simulink model "Simulaciones_de_Control"  (R2026b)
settings: Solver=ode15s  StopTime=3  MaxStep=1e-3
values from neighbouring files (symbols this model uses):
  alpha_Cu = 3.9e-3    (= 0.0039)    [coeficientes.m]
  b_eq = b_m + b_l/(r^2)    (= 2.19444444444e-05)    [coeficientes.m]
  C_ts = 0.818    [coeficientes.m]
  g = 9.80665    [coeficientes.m]
  init_I0 = 0    [coeficientes.m]
  init_Id = 0    [coeficientes.m]
  init_Iq = 0    [coeficientes.m]
  init_theta = 0    [coeficientes.m]
  init_Ts = 20    [coeficientes.m]
  init_w = 0    [coeficientes.m]
  J_eq = J_m + J_l/(r^2)    (= 4.58263888889e-05)    [coeficientes.m]
  K_et = 2*p_obs    (= 6400)    [coeficientes.m]
  K_ew = p_obs^2    (= 10240000)    [coeficientes.m]
  k_l = k_l_min + m_l*l_l    (= 1)    [coeficientes.m]
  Kd_mov = wn_mov * (2*zeta_mov + 1) * J_eq    (= 0.0916527777778)    [coeficientes.m]
  Ki_mov = wn_mov^3 * J_eq    (= 23463.1111111)    [coeficientes.m]
  Kp_mov = wn_mov^2 * (2*zeta_mov + 1) * J_eq    (= 73.3222222222)    [coeficientes.m]
  L_d = 6.6e-3    (= 0.0066)    [coeficientes.m]
  L_ls = 0.8e-3    (= 0.0008)    [coeficientes.m]
  L_q = 5.8e-3    (= 0.0058)    [coeficientes.m]
  lambda = 0.016    [coeficientes.m]
  Pp = 3    [coeficientes.m]
  r = 120.0    (= 120)    [coeficientes.m]
  R_sREF = 1.02    [coeficientes.m]
  R_tsamb = 146.7    [coeficientes.m]
  T_amb = 20    [coeficientes.m]
  T_sREF = 20    [coeficientes.m]
libraries: eeTransforms x12
(part 1 of 2)
settings Model: Creator=fedeb  LastModifiedBy=fedeb
settings SimscapeCC: SimscapeLogType=all  SimscapeNominalValues="[{\"value\":\"1\",\"unit\":\"A\"},{\"value\":\"1\",\"unit\":\"bar\"},{\"value\":\"1\",\"unit\":\"cm^2\"},{\"value\":\"1\",\"unit\":\"cm^3/s\"},{\"value\":\"1\",\"unit\":\"kJ/kg\"},{\"value\":\"1\",\"unit\":\"kW\"},{\"value\":\"1\",\"unit\":\"l\"},{\"value\":\"1\",\"unit\":\"N\"},{\"value\":\"1\",\"unit\":\"N*m\"},{\"value\":\"1\",\"unit\":\"V\"},{\"value\":\"0.001\",\"unit\":\"Wb\"}]"  SimscapeUseEnergyAccounting=off

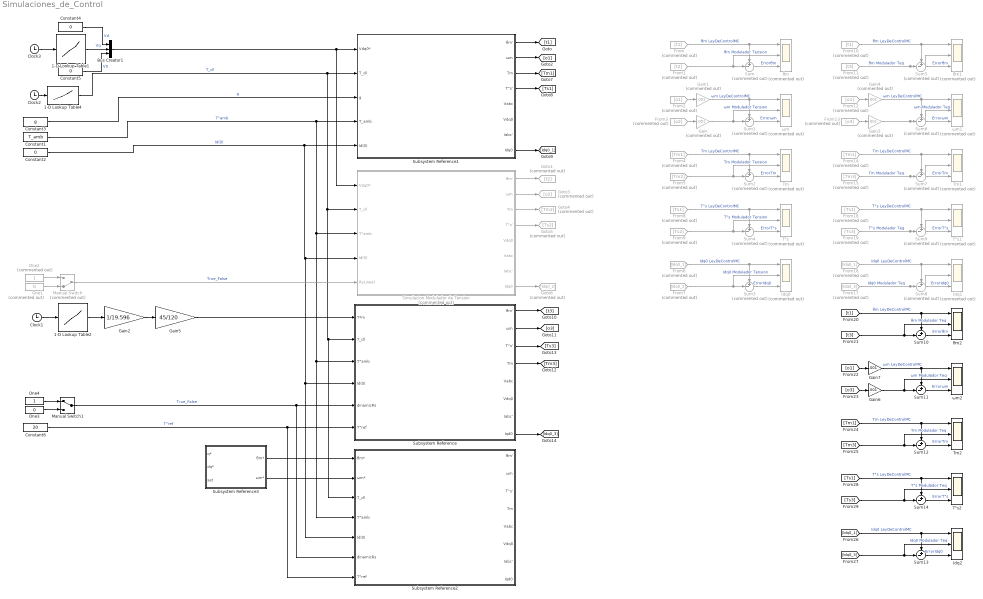
== system Simulaciones_de_Control ==
  1-D Lookup Table1 : Lookup_n-D  NumberOfTableDimensions=1  BreakpointsForDimension1=[0.0, 0.1, 0.101, 0.3, 0.301, 0.5, 0.501, 0.7, 0.701, 0.9, 0.901, 1.1, 1.101, 1.3, 1.301, 1.5, 1.501, 1.7, 1.701, 1.9, 1.901, 2.0]  Table=[0.0, 0.0, 19.596, 19.596, 19.596, 19.596, 19.596, 19.596, 0.0, 0.0, 0.0, 0.0, -19.596, -19.596, -19.596, -19.596, -19.596, -19.596, 0.0, 0.0, 0.0, 0.0]  InternalRulePriority=Speed  RndMeth=Simplest
  1-D Lookup Table2 : Lookup_n-D  NumberOfTableDimensions=1  BreakpointsForDimension1=[0.0, 0.1, 0.101, 0.3, 0.301, 0.5, 0.501, 0.7, 0.701, 0.9, 0.901, 1.1, 1.101, 1.3, 1.301, 1.5, 1.501, 1.7, 1.701, 1.9, 1.901, 2.0]  Table=[0.0, 0.0, 19.596, 19.596, 19.596, 19.596, 19.596, 19.596, 0.0, 0.0, 0.0, 0.0, -19.596, -19.596, -19.596, -19.596, -19.596, -19.596, 0.0, 0.0, 0.0, 0.0]  InternalRulePriority=Speed  RndMeth=Simplest
  1-D Lookup Table4 : Lookup_n-D  NumberOfTableDimensions=1  BreakpointsForDimension1=[0.0, 0.1, 0.101, 0.3, 0.301, 0.5, 0.501, 0.7, 0.701, 0.9, 0.901, 1.1, 1.101, 1.3, 1.301, 1.5, 1.501, 1.7, 1.701, 1.9, 1.901, 2.0]  Table=[0.0, 0.0, 0.0, 0.0, 6.28, 6.28, -6.28, -6.28, -6.28, -6.28, 0.0, 0.0, 0.0, 0.0, 6.28, 6.28, -6.28, -6.28, 0.0, 0.0, 0.0, 0.0]  InternalRulePriority=Speed  RndMeth=Simplest
  Bus Creator1 : BusCreator  Inputs=3
  Clock1 : Clock
  Clock2 : Clock
  Clock3 : Clock
  Constant1 : Constant  Value=T_amb
  Constant2 : Constant  Value=0
  Constant3 : Constant  Value=g
  Constant4 : Constant  Value=0
  Constant5 : Constant  Value=0
  Constant6 : Constant  Value=20
  From : From  Commented=on  GotoTag=t1
  From1 : From  Commented=on  GotoTag=t2
  From10 : From  Commented=on  GotoTag=t1
  From11 : From  Commented=on  GotoTag=t3
  From12 : From  Commented=on  GotoTag=o1
  From13 : From  Commented=on  GotoTag=o3
  From14 : From  Commented=on  GotoTag=Tm1
  From15 : From  Commented=on  GotoTag=Tm3
  From16 : From  Commented=on  GotoTag=Idq0_1
  From17 : From  Commented=on  GotoTag=Idq0_3
  From18 : From  Commented=on  GotoTag=Ts1
  From19 : From  Commented=on  GotoTag=Ts3
  From2 : From  Commented=on  GotoTag=o1
  From3 : From  Commented=on  GotoTag=o2
  From4 : From  Commented=on  GotoTag=Tm1
  From5 : From  Commented=on  GotoTag=Tm2
  From6 : From  Commented=on  GotoTag=Idq0_1
  From7 : From  Commented=on  GotoTag=Idq0_2
  From8 : From  Commented=on  GotoTag=Ts1
  From9 : From  Commented=on  GotoTag=Ts2
  Gain{,1,3..4} (4 alike) : Gain  Commented=on  Gain=.001
  Gain2 : Gain  Gain=1/19.596
  Gain5 : Gain  Gain=45/120
  Gain6 : Gain  Gain=.001
  Gain7 : Gain  Gain=.001
  Goto1 : Goto  Commented=on  GotoTag=t2
  Goto3 : Goto  Commented=on  GotoTag=o2
  Goto4 : Goto  Commented=on  GotoTag=Tm2
  Goto5 : Goto  Commented=on  GotoTag=Ts2
  Goto6 : Goto  Commented=on  GotoTag=Idq0_2
  Idq0 : Scope  Commented=on  NumInputPorts=3
      settings: Title=Comparación Idq0  ActiveDisplayYMinimum=-22.799596876170931  ActiveDisplayYMaximum=77.542210763995357  YLabel=Idq0 [A]  DataLoggingVariableName=ScopeData3
  Idq1 : Scope  Commented=on  NumInputPorts=3
      settings: Title=Comparación Idq0  ActiveDisplayYMinimum=-15.292921358243067  ActiveDisplayYMaximum=15.917825301373405  YLabel=Idq0 [A]  DataLoggingVariableName=ScopeData4
  Idq2 : Scope  NumInputPorts=3
      settings: Title=Comparación Idq0  ActiveDisplayYMinimum=-15.292921358243067  ActiveDisplayYMaximum=15.917825301373405  YLabel=Idq0 [A]  DataLoggingVariableName=ScopeData10
  Manual Switch : ManualSwitch  Commented=on  CurrentSetting=0
  Manual Switch1 : ManualSwitch
  One1 : Constant  Commented=on  Value=0  OutDataTypeStr=Inherit: Inherit via back propagation
  One2 : Constant  Commented=on  OutDataTypeStr=Inherit: Inherit via back propagation
  One3 : Constant  Value=0  OutDataTypeStr=Inherit: Inherit via back propagation
  One4 : Constant  OutDataTypeStr=Inherit: Inherit via back propagation
  Simulacion Modulador de Tension : Subsystem  Commented=on
  Subsystem Reference : Subsystem
  Subsystem Reference1 : Subsystem
  Subsystem Reference2 : Subsystem
  Subsystem Reference3 : Subsystem
  Sum{,1..9} (10 alike) : Sum  Commented=on  Inputs=+-|
  Sum{10..14} (5 alike) : Sum  Inputs=+-|
  Tm : Scope  Commented=on  NumInputPorts=3
      settings: Title=Comparación Torque Motor  ActiveDisplayYMinimum=-1.641570975092526  ActiveDisplayYMaximum=5.5830391750086239  YLabel=T_m [Nm]
  Tm1 : Scope  Commented=on  NumInputPorts=3
      settings: Title=Comparación Torque Motor  ActiveDisplayYMinimum=-1.1010903377934618  ActiveDisplayYMaximum=1.1460834216988809  YLabel=T_m [Nm]  DataLoggingVariableName=ScopeData6
  Tm2 : Scope  NumInputPorts=3
      settings: Title=Comparación Torque Motor  ActiveDisplayYMinimum=-1.1010903377934618  ActiveDisplayYMaximum=1.1460834216988809  YLabel=T_m [Nm]  DataLoggingVariableName=ScopeData11
  T°s : Scope  Commented=on  NumInputPorts=3
      settings: Title=Comparación θm  ActiveDisplayYMinimum=-1017.2983087504352  ActiveDisplayYMaximum=1033.0305039187574  DataLoggingVariableName=ScopeData2
  T°s1 : Scope  Commented=on  NumInputPorts=3
      settings: Title=Comparación T°s  ActiveDisplayYMinimum=10.145079259650506  ActiveDisplayYMaximum=108.69428666314548  YLabel=T°s [°C]  DataLoggingVariableName=ScopeData7
  T°s2 : Scope  NumInputPorts=3
      settings: Title=Comparación T°s  ActiveDisplayYMinimum=10.145079259650506  ActiveDisplayYMaximum=108.69428666314548  YLabel=T°s [°C]  DataLoggingVariableName=ScopeData12
  θm : Scope  Commented=on  NumInputPorts=3
      settings: Title=Comparación θm  ActiveDisplayYMinimum=-15548.638838676963  ActiveDisplayYMaximum=15530.228334297437
  θm1 : Scope  Commented=on  NumInputPorts=3
      settings: Title=Comparación θm  ActiveDisplayYMinimum=-693.83102797369031  ActiveDisplayYMaximum=5988.9336809294882  YLabel=\theta_m [rad]  DataLoggingVariableName=ScopeData8
  θm2 : Scope  NumInputPorts=3
      settings: Title=Comparación θm  ActiveDisplayYMinimum=-693.83102797369031  ActiveDisplayYMaximum=5988.9336809294882  YLabel=\theta_m [rad]  DataLoggingVariableName=ScopeData13
  ωm : Scope  Commented=on  NumInputPorts=3
      settings: Title=Comparación ωm  ActiveDisplayYMinimum=-1.8612728525157345  ActiveDisplayYMaximum=12.323556548165303  YLabel=\omega_{motor} [10^3 rad/s]  DataLoggingVariableName=ScopeData5
  ωm1 : Scope  Commented=on  NumInputPorts=3
      settings: Title=Comparación ωm  ActiveDisplayYMinimum=-1.1427898971415431  ActiveDisplayYMaximum=5.8360821110076726  YLabel=\omega_{motor} [10^3 rad/s]  DataLoggingVariableName=ScopeData9
  ωm2 : Scope  NumInputPorts=3
      settings: Title=Comparación ωm  ActiveDisplayYMinimum=-1.1427898971415431  ActiveDisplayYMaximum=5.8360821110076726  YLabel=\omega_{motor} [10^3 rad/s]  DataLoggingVariableName=ScopeData14
  wires:
  Clock3/1 -> 1-D Lookup Table1/1
  1-D Lookup Table1/1 -> Bus Creator1/2  "Vq"
  Clock2/1 -> 1-D Lookup Table4/1
  Constant5/1 -> Bus Creator1/3  "V0"
  Constant4/1 -> Bus Creator1/1  "Vd"
  1-D Lookup Table4/1 -> Subsystem Reference2/3(T_dl), Subsystem Reference/2(T_dl), Simulacion Modulador de Tension/2(T_dl), Subsystem Reference1/2(T_dl)  "T_dl"
  Bus Creator1/1 -> Simulacion Modulador de Tension/1(Vdq0*), Subsystem Reference1/1(Vdq0*)
  Constant3/1 -> Subsystem Reference1/3(g)  "g"
  Constant1/1 -> Subsystem Reference2/4(T°amb), Subsystem Reference/3(T°amb), Simulacion Modulador de Tension/3(T°amb), Subsystem Reference1/4(T_amb)  "T°amb"
  Constant2/1 -> Subsystem Reference2/5(Id(0)), Subsystem Reference/4(Id(0)), Simulacion Modulador de Tension/4(Id(0)), Subsystem Reference1/5(Id(0))  "Id(0)"
  One2/1 -> Manual Switch/1
  One1/1 -> Manual Switch/2
  Manual Switch/1 -> Simulacion Modulador de Tension/5(RsLineal)  "True_False"
  Sum/1 -> θm/3  "Errorθm"
  Subsystem Reference1/1(θm') -> [t1]
  From/1 -> θm/1, Sum/1  "θm LeyDeControlMC"
  Simulacion Modulador de Tension/1(θm') -> Goto1/1
  From1/1 -> θm/2, Sum/2  "θm Modulador Tension"
  From3/1 -> Gain/1
  Sum1/1 -> ωm/3  "Errorωm"
  From2/1 -> Gain1/1
  From5/1 -> Tm/2, Sum2/2  "Tm Modulador Tension"
  Sum2/1 -> Tm/3  "ErrorTm"
  From4/1 -> Tm/1, Sum2/1  "Tm LeyDeControlMC"
  From7/1 -> Idq0/2, Sum3/2  "Idq0 Modulador Tension"
  Sum3/1 -> Idq0/3  "ErrorIdq0"
  From6/1 -> Idq0/1, Sum3/1  "Idq0 LeyDeControlMC"
  Subsystem Reference1/2(ωm) -> [o1]
  Subsystem Reference1/3(Tm) -> [Tm1]
  Subsystem Reference1/4(T°s') -> [Ts1]
  Subsystem Reference1/8(Idq0) -> [Idq0_1]
  Simulacion Modulador de Tension/2(ωm) -> Goto3/1
  Simulacion Modulador de Tension/3(Tm) -> Goto4/1
  Simulacion Modulador de Tension/4(T°s') -> Goto5/1
  Simulacion Modulador de Tension/8(Idq0) -> Goto6/1
  From8/1 -> T°s/1, Sum4/1  "T°s LeyDeControlMC"
  Sum4/1 -> T°s/3  "ErrorT°s"
  From9/1 -> T°s/2, Sum4/2  "T°s Modulador Tension"
  Gain/1 -> ωm/2, Sum1/2  "ωm Modulador Tension"
  Gain1/1 -> ωm/1, Sum1/1  "ωm LeyDeControlMC"
  Subsystem Reference/1(θm') -> [t3]
  Clock1/1 -> 1-D Lookup Table2/1
  1-D Lookup Table2/1 -> Gain2/1
  Gain2/1 -> Gain5/1
  One4/1 -> Manual Switch1/1
  One3/1 -> Manual Switch1/2
  Manual Switch1/1 -> Subsystem Reference2/6(dinamicRs), Subsystem Reference/5(dinamicRs)  "True_False"
  Constant6/1 -> Subsystem Reference2/7(T°ref), Subsystem Reference/6(T°ref)  "T°ref"
  Subsystem Reference/2(ωm) -> [o3]
  Subsystem Reference/3(T°s') -> [Ts3]
  Subsystem Reference/4(Tm) -> [Tm3]
  Subsystem Reference/8(Iqd0) -> [Idq0_3]
  Sum9/1 -> T°s1/3  "ErrorT°s"
  Sum6/1 -> ωm1/3  "Errorωm"
  From16/1 -> Idq1/1, Sum8/1  "Idq0 LeyDeControlMC"
  From19/1 -> T°s1/2, Sum9/2  "T°s Modulador Teq"
  Gain3/1 -> ωm1/2, Sum6/2  "ωm Modulador Teq"
  From14/1 -> Tm1/1, Sum7/1  "Tm LeyDeControlMC"
  Gain4/1 -> ωm1/1, Sum6/1  "ωm LeyDeControlMC"
  Sum7/1 -> Tm1/3  "ErrorTm"
  From17/1 -> Idq1/2, Sum8/2  "Idq0 Modulador Teq"
  Sum8/1 -> Idq1/3  "ErrorIdq0"
  From12/1 -> Gain4/1
  From11/1 -> θm1/2, Sum5/2  "θm Modulador Teq"
  From18/1 -> T°s1/1, Sum9/1  "T°s LeyDeControlMC"
  Sum5/1 -> θm1/3  "Errorθm"
  From10/1 -> θm1/1, Sum5/1  "θm LeyDeControlMC"
  From13/1 -> Gain3/1
  From15/1 -> Tm1/2, Sum7/2  "Tm Modulador Teq"
  Gain5/1 -> Subsystem Reference/1(T*m)
  [Idq0_1] -> Idq2/1, Sum13/1  "Idq0 LeyDeControlMC"
  [Ts3] -> T°s2/2, Sum14/2  "T°s Modulador Teq"
  Sum10/1 -> θm2/3  "Errorθm"
  [t1] -> θm2/1, Sum10/1  "θm LeyDeControlMC"
  Sum14/1 -> T°s2/3  "ErrorT°s"
  [Idq0_3] -> Idq2/2, Sum13/2  "Idq0 Modulador Teq"
  Sum11/1 -> ωm2/3  "Errorωm"
  [t3] -> θm2/2, Sum10/2  "θm Modulador Teq"
  Sum12/1 -> Tm2/3  "ErrorTm"
  [Ts1] -> T°s2/1, Sum14/1  "T°s LeyDeControlMC"
  [Tm1] -> Tm2/1, Sum12/1  "Tm LeyDeControlMC"
  Gain7/1 -> ωm2/1, Sum11/1  "ωm LeyDeControlMC"
  [Tm3] -> Tm2/2, Sum12/2  "Tm Modulador Teq"
  [o1] -> Gain7/1
  Gain6/1 -> ωm2/2, Sum11/2  "ωm Modulador Teq"
  [o3] -> Gain6/1
  Sum13/1 -> Idq2/3  "ErrorIdq0"
  Subsystem Reference3/2(ωm*) -> Subsystem Reference2/2(ωm*)
  Subsystem Reference3/1(θm*) -> Subsystem Reference2/1(θm*)

== system Simulaciones_de_Control/Simulacion Modulador de Tension ==
  Vdq0* : Inport  OutDataTypeStr=Bus: Vdq0
  T_dl : Inport  Port=2
  T°amb : Inport  Port=3
  Id(0) : Inport  Port=4
  RsLineal : Inport  Port=5
  Bus Selector2 : BusSelector  OutputSignals=Vd,Vq,V0
  Constant : Constant  Value=g
  Constant2 : Constant  Value=R_sREF
  Modulador de Tensiones Virtuales : Subsystem
      settings: PortSchema="{\"entries\":[{\"content\":{\"sides\":[{\"content\":{\"connectorIds\":[\"In2\",\"In1\",\"In3\",\"In6\",\"In7\",\"In5\",\"In4\"]},\"type\":\"ConnectorPlacement.EquallySpacedRectSide\",\"uuid\":\"561a625a-719f-47d4-85d3-a88e423068dd\"},{\"content\":{\"connectorIds\":[\"Out2\",\"Out1\"],\"side\":\"RIGHT\"},\"type\":\"ConnectorPlacement.EquallySpacedRectSide\",\"uuid\":\"c1cdd74a-6c1d-470e-a6ac-8d72e83b5cc5\"},{\"content\":{\"side\":\"TOP\"},\"type\":\"ConnectorPlacement.EquallySpacedRectSide\",\"uuid\":\"c5935c6f-534c-46b9-aa64-6d6dabbbb210\"}]},\"type\":\"ConnectorPlacement.EquallySpacedConnector\",\"uuid\":\"b0debde9-6e18-4e06-b0c4-28c9c51e472d\"}],\"packageUris\":[\"http://schema.mathworks.com/mf0/Connector/R2020b\"],\"version\":\"1.0\"}"
  Planta (Modelo Global No Lineal) : Subsystem
      settings: PortSchema="{\"entries\":[{\"content\":{\"sides\":[{\"content\":{\"connectorIds\":[\"In1\",\"In3\",\"In2\",\"In4\",\"In5\"]},\"type\":\"ConnectorPlacement.EquallySpacedRectSide\",\"uuid\":\"3481abf0-b0cb-49f6-b93f-5a31fbfa4119\"},{\"content\":{\"connectorIds\":[\"Out1\",\"Out2\",\"Out3\",\"Out4\",\"Out5\"],\"side\":\"RIGHT\"},\"type\":\"ConnectorPlacement.EquallySpacedRectSide\",\"uuid\":\"81dbc61e-d5f3-4edc-bc73-ec3d6160a008\"},{\"content\":{\"side\":\"TOP\"},\"type\":\"ConnectorPlacement.EquallySpacedRectSide\",\"uuid\":\"48e37594-92fb-4835-b4aa-9211b8b6a309\"}]},\"type\":\"ConnectorPlacement.EquallySpacedConnector\",\"uuid\":\"6c32b8e1-5803-41f4-af4e-ba3a494349ba\"}],\"packageUris\":[\"http://schema.mathworks.com/mf0/Connector/R2020b\"],\"version\":\"1.0\"}"
  Sensores Ideales : Subsystem
      settings: PortSchema="{\"entries\":[{\"content\":{\"sides\":[{\"content\":{\"connectorIds\":[\"In1\",\"In2\",\"In3\"]},\"type\":\"ConnectorPlacement.EquallySpacedRectSide\",\"uuid\":\"f4bb6189-c8cb-4d3e-a45f-895d59b6a7f9\"},{\"content\":{\"connectorIds\":[\"Out3\",\"Out2\",\"Out1\"],\"side\":\"RIGHT\"},\"type\":\"ConnectorPlacement.EquallySpacedRectSide\",\"uuid\":\"4fe23da4-d7b3-4116-8a5c-3a889a14c1ed\"},{\"content\":{\"side\":\"TOP\"},\"type\":\"ConnectorPlacement.EquallySpacedRectSide\",\"uuid\":\"3a675bb7-2a54-45fb-91cd-5f3dc1d0d742\"}]},\"type\":\"ConnectorPlacement.EquallySpacedConnector\",\"uuid\":\"fa703284-8060-4ab8-a349-fe5cb05f502a\"}],\"packageUris\":[\"http://schema.mathworks.com/mf0/Connector/R2020b\"],\"version\":\"1.0\"}"
  Subsystem : Subsystem
  Switch : Switch  Criteria=u2 > Threshold  SaturateOnIntegerOverflow=off  InputSameDT=off
  Transformada_Directa_de_Park_I : Subsystem
  θm' : Outport
  ωm : Outport  Port=2
  Tm : Outport  Port=3
  T°s' : Outport  Port=4
  Vdq0 : Outport  Port=5
  Vabc : Outport  Port=6
  Iabc' : Outport  Port=7
  Idq0 : Outport  Port=8  OutDataTypeStr=Bus: Idq0
  wires:
  Planta (Modelo Global No Lineal)/5(Tm) -> Tm/1
  Id(0)/1 -> Planta (Modelo Global No Lineal)/5(Id(0))
  T_dl/1 -> Planta (Modelo Global No Lineal)/2(T_ld)
  Modulador de Tensiones Virtuales/2(Vdq0) -> Vdq0/1
  Planta (Modelo Global No Lineal)/3(T°s) -> Sensores Ideales/3(T°s)
  Sensores Ideales/2(Iabc') -> Transformada_Directa_de_Park_I/1(Iabc), Modulador de Tensiones Virtuales/6(Iabc), Iabc'/1  "Iabc'"
  T°amb/1 -> Planta (Modelo Global No Lineal)/4(T°amb)
  Constant/1 -> Planta (Modelo Global No Lineal)/3(g)
  Planta (Modelo Global No Lineal)/1(θm) -> Sensores Ideales/1(θm)
  Modulador de Tensiones Virtuales/1(Vabc) -> Vabc/1, Planta (Modelo Global No Lineal)/1(Vabc)
  Sensores Ideales/3(T°s') -> Subsystem/1(T°s), T°s'/1  "T°s'"
  Sensores Ideales/1(θm') -> Transformada_Directa_de_Park_I/2(θm), Modulador de Tensiones Virtuales/7(θm), θm'/1  "θm'"
  Planta (Modelo Global No Lineal)/2(Iabc) -> Sensores Ideales/2(Iabc)
  Planta (Modelo Global No Lineal)/4(ωm) -> Modulador de Tensiones Virtuales/5(ωm), ωm/1  "ωm"
  Subsystem/1(R_s) -> Switch/1  "Rs"
  RsLineal/1 -> Switch/2  "True_False"
  Switch/1 -> Modulador de Tensiones Virtuales/4(Rs)  "Rs"
  Constant2/1 -> Switch/3
  Transformada_Directa_de_Park_I/1(Idq0) -> Idq0/1
  Bus Selector2/1 -> Modulador de Tensiones Virtuales/2(Vd*)  "<Vd>"
  Bus Selector2/3 -> Modulador de Tensiones Virtuales/3(V0*)  "<V0>"
  Bus Selector2/2 -> Modulador de Tensiones Virtuales/1(Vq*)  "<Vq>"
  Vdq0*/1 -> Bus Selector2/1

== system Simulaciones_de_Control/Subsystem Reference ==
  T*m : Inport
  T_dl : Inport  Port=2
  T°amb : Inport  Port=3
  Id(0) : Inport  Port=4
  dinamicRs : Inport  Port=5
  T°ref : Inport  Port=6
  Constant : Constant  Value=g
  Modulador de Torque Equivalente : Subsystem
      settings: PortSchema="{\"entries\":[{\"content\":{\"sides\":[{\"content\":{\"connectorIds\":[\"In1\",\"In3\",\"In5\",\"In2\",\"In4\",\"In6\",\"In7\"]},\"type\":\"ConnectorPlacement.EquallySpacedRectSide\",\"uuid\":\"ea9ad4ab-f607-4d37-9442-85f6cfda2486\"},{\"content\":{\"connectorIds\":[\"Out2\",\"Out1\"],\"side\":\"RIGHT\"},\"type\":\"ConnectorPlacement.EquallySpacedRectSide\",\"uuid\":\"696b5fe5-1f6c-4fc9-932e-86b56d49996f\"},{\"content\":{\"side\":\"TOP\"},\"type\":\"ConnectorPlacement.EquallySpacedRectSide\",\"uuid\":\"45e3ac4c-5a2f-4a79-9454-e497b07295c7\"}]},\"type\":\"ConnectorPlacement.EquallySpacedConnector\",\"uuid\":\"ad401c21-3c60-4ab4-96eb-f449fc93609a\"}],\"packageUris\":[\"http://schema.mathworks.com/mf0/Connector/R2020b\"],\"version\":\"1.0\"}"
  Planta (Modelo Global No Lineal) : Subsystem
      settings: PortSchema="{\"entries\":[{\"content\":{\"sides\":[{\"content\":{\"connectorIds\":[\"In1\",\"In3\",\"In2\",\"In4\",\"In5\"]},\"type\":\"ConnectorPlacement.EquallySpacedRectSide\",\"uuid\":\"3481abf0-b0cb-49f6-b93f-5a31fbfa4119\"},{\"content\":{\"connectorIds\":[\"Out1\",\"Out2\",\"Out3\",\"Out4\",\"Out5\"],\"side\":\"RIGHT\"},\"type\":\"ConnectorPlacement.EquallySpacedRectSide\",\"uuid\":\"81dbc61e-d5f3-4edc-bc73-ec3d6160a008\"},{\"content\":{\"side\":\"TOP\"},\"type\":\"ConnectorPlacement.EquallySpacedRectSide\",\"uuid\":\"48e37594-92fb-4835-b4aa-9211b8b6a309\"}]},\"type\":\"ConnectorPlacement.EquallySpacedConnector\",\"uuid\":\"6c32b8e1-5803-41f4-af4e-ba3a494349ba\"}],\"packageUris\":[\"http://schema.mathworks.com/mf0/Connector/R2020b\"],\"version\":\"1.0\"}"
  Sensores Ideales : Subsystem
      settings: PortSchema="{\"entries\":[{\"content\":{\"sides\":[{\"content\":{\"connectorIds\":[\"In1\",\"In2\",\"In3\"]},\"type\":\"ConnectorPlacement.EquallySpacedRectSide\",\"uuid\":\"f4bb6189-c8cb-4d3e-a45f-895d59b6a7f9\"},{\"content\":{\"connectorIds\":[\"Out3\",\"Out2\",\"Out1\"],\"side\":\"RIGHT\"},\"type\":\"ConnectorPlacement.EquallySpacedRectSide\",\"uuid\":\"4fe23da4-d7b3-4116-8a5c-3a889a14c1ed\"},{\"content\":{\"side\":\"TOP\"},\"type\":\"ConnectorPlacement.EquallySpacedRectSide\",\"uuid\":\"3a675bb7-2a54-45fb-91cd-5f3dc1d0d742\"}]},\"type\":\"ConnectorPlacement.EquallySpacedConnector\",\"uuid\":\"fa703284-8060-4ab8-a349-fe5cb05f502a\"}],\"packageUris\":[\"http://schema.mathworks.com/mf0/Connector/R2020b\"],\"version\":\"1.0\"}"
  Transformada_Directa_de_Park_I : Subsystem
  θm' : Outport
  ωm : Outport  Port=2
  T°s' : Outport  Port=3
  Tm : Outport  Port=4
  Vabc : Outport  Port=5  OutDataTypeStr=Bus: Vabc
  Vdq0 : Outport  Port=6  OutDataTypeStr=Bus: Vdq0
  Iabc' : Outport  Port=7  OutDataTypeStr=Bus: Iabc
  Iqd0 : Outport  Port=8  OutDataTypeStr=Bus: Idq0
  wires:
  Planta (Modelo Global No Lineal)/1(θm) -> Sensores Ideales/1(θm)
  Sensores Ideales/1(θm') -> θm'/1, Transformada_Directa_de_Park_I/2(θm), Modulador de Torque Equivalente/4(θm)  "θm'"
  Planta (Modelo Global No Lineal)/2(Iabc) -> Sensores Ideales/2(Iabc)
  Modulador de Torque Equivalente/1(Vabc) -> Planta (Modelo Global No Lineal)/1(Vabc), Vabc/1
  Planta (Modelo Global No Lineal)/3(T°s) -> Sensores Ideales/3(T°s)
  Sensores Ideales/2(Iabc') -> Transformada_Directa_de_Park_I/1(Iabc), Modulador de Torque Equivalente/3(Iabc), Iabc'/1  "Iabc'"
  Sensores Ideales/3(T°s') -> T°s'/1, Modulador de Torque Equivalente/1(T°s)  "T°s'"
  Constant/1 -> Planta (Modelo Global No Lineal)/3(g)
  Id(0)/1 -> Planta (Modelo Global No Lineal)/5(Id(0))  "Id(0)"
  T°amb/1 -> Planta (Modelo Global No Lineal)/4(T°amb)  "T°amb"
  T_dl/1 -> Planta (Modelo Global No Lineal)/2(T_ld)  "T_dl"
  Planta (Modelo Global No Lineal)/5(Tm) -> Tm/1
  Planta (Modelo Global No Lineal)/4(ωm) -> Modulador de Torque Equivalente/2(ωm), ωm/1
  Modulador de Torque Equivalente/2(Vdq0) -> Vdq0/1
  dinamicRs/1 -> Modulador de Torque Equivalente/6(dinamicRs?)
  T°ref/1 -> Modulador de Torque Equivalente/7(T°ref)
  T*m/1 -> Modulador de Torque Equivalente/5(T*m)  "T*m"
  Transformada_Directa_de_Park_I/1(Idq0) -> Iqd0/1

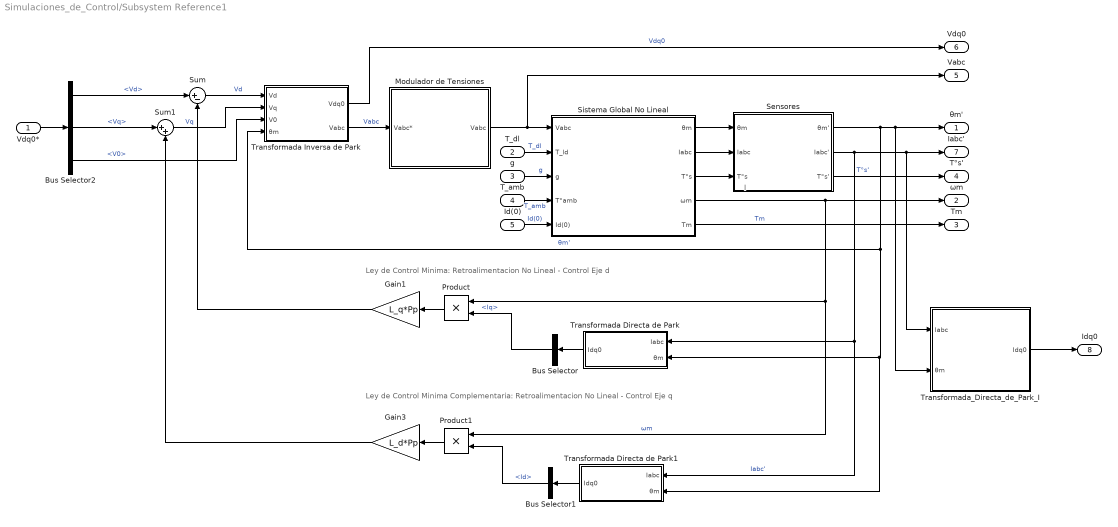
== system Simulaciones_de_Control/Subsystem Reference1 ==
  note: Ley de Control Minima: Retroalimentacion No Lineal - Control Eje d
  note: I
  note: Ley de Control Minima Complementaria: Retroalimentacion No Lineal - Control Eje q
  Vdq0* : Inport  OutDataTypeStr=Bus: Vdq0
  T_dl : Inport  Port=2
  g : Inport  Port=3
  T_amb : Inport  Port=4
  Id(0) : Inport  Port=5
  Bus Selector : BusSelector  OutputSignals=Iq
  Bus Selector1 : BusSelector  OutputSignals=Id
  Bus Selector2 : BusSelector  OutputSignals=Vd,Vq,V0
  Gain1 : Gain  Gain=L_q*Pp
  Gain3 : Gain  Gain=L_d*Pp
  Modulador de Tensiones : Subsystem
  Product : Product
  Product1 : Product
  Sensores : Subsystem
  Sistema Global No Lineal : Subsystem
  Sum : Sum  Inputs=|+-
  Sum1 : Sum  Inputs=|++
  Transformada Directa de Park : Subsystem
  Transformada Directa de Park1 : Subsystem
  Transformada Inversa de Park : Subsystem
      settings: PortSchema="{\"entries\":[{\"content\":{\"sides\":[{\"content\":{\"connectorIds\":[\"In2\",\"In3\",\"In4\",\"In1\"]},\"type\":\"ConnectorPlacement.EquallySpacedRectSide\",\"uuid\":\"6292945e-98e2-47d0-b051-6efca1f5a94c\"},{\"content\":{\"connectorIds\":[\"Out1\",\"Out2\"],\"side\":\"RIGHT\"},\"type\":\"ConnectorPlacement.EquallySpacedRectSide\",\"uuid\":\"7de8e65d-1a52-4b6e-b95f-22e2aa3d5ce9\"},{\"content\":{\"side\":\"TOP\"},\"type\":\"ConnectorPlacement.EquallySpacedRectSide\",\"uuid\":\"f4a26ab7-c226-4517-988b-56c9287c32f3\"}]},\"type\":\"ConnectorPlacement.EquallySpacedConnector\",\"uuid\":\"2fa12274-dda1-4d9d-bdf4-02dff97f265b\"}],\"packageUris\":[\"http://schema.mathworks.com/mf0/Connector/R2020b\"],\"version\":\"1.0\"}"
  Transformada_Directa_de_Park_I : Subsystem
  θm' : Outport
  ωm : Outport  Port=2
  Tm : Outport  Port=3
  T°s' : Outport  Port=4
  Vabc : Outport  Port=5  OutDataTypeStr=Bus: Vabc
  Vdq0 : Outport  Port=6  OutDataTypeStr=Bus: Vdq0
  Iabc' : Outport  Port=7  OutDataTypeStr=Bus: Iabc
  Idq0 : Outport  Port=8  OutDataTypeStr=Bus: Idq0
  wires:
  Sistema Global No Lineal/3(T°s) -> Sensores/3(T°s)
  Bus Selector/1 -> Product/2  "<Iq>"
  T_dl/1 -> Sistema Global No Lineal/2(T_ld)  "T_dl"
  Bus Selector2/2 -> Sum1/1  "<Vq>"
  Sensores/1(θm') -> Transformada Inversa de Park/1(θm), Transformada Directa de Park/2(θm), Transformada Directa de Park1/2(θm), Transformada_Directa_de_Park_I/2(θm), θm'/1  "θm'"
  Gain1/1 -> Sum/2
  Sum/1 -> Transformada Inversa de Park/2(Vd)  "Vd"
  Sensores/3(T°s') -> T°s'/1  "T°s'"
  Sum1/1 -> Transformada Inversa de Park/3(Vq)  "Vq"
  Bus Selector1/1 -> Product1/2  "<Id>"
  Id(0)/1 -> Sistema Global No Lineal/5(Id(0))  "Id(0)"
  Sistema Global No Lineal/5(Tm) -> Tm/1  "Tm"
  Transformada Inversa de Park/1(Vdq0) -> Vdq0/1  "Vdq0"
  Bus Selector2/3 -> Transformada Inversa de Park/4(V0)  "<V0>"
  Transformada Inversa de Park/2(Vabc) -> Modulador de Tensiones/1(Vabc*)  "Vabc"
  g/1 -> Sistema Global No Lineal/3(g)  "g"
  Sistema Global No Lineal/1(θm) -> Sensores/1(θm)
  Transformada Directa de Park/1(Idq0) -> Bus Selector/1
  T_amb/1 -> Sistema Global No Lineal/4(T°amb)  "T_amb"
  Sistema Global No Lineal/2(Iabc) -> Sensores/2(Iabc)
  Sistema Global No Lineal/4(ωm) -> Product/1, Product1/1, ωm/1  "ωm"
  Product/1 -> Gain1/1
  Product1/1 -> Gain3/1
  Bus Selector2/1 -> Sum/1  "<Vd>"
  Modulador de Tensiones/1(Vabc) -> Vabc/1, Sistema Global No Lineal/1(Vabc)
  Transformada Directa de Park1/1(Idq0) -> Bus Selector1/1
  Sensores/2(Iabc') -> Transformada_Directa_de_Park_I/1(Iabc), Iabc'/1, Transformada Directa de Park/1(Iabc), Transformada Directa de Park1/1(Iabc)  "Iabc'"
  Gain3/1 -> Sum1/2
  Vdq0*/1 -> Bus Selector2/1
  Transformada_Directa_de_Park_I/1(Idq0) -> Idq0/1

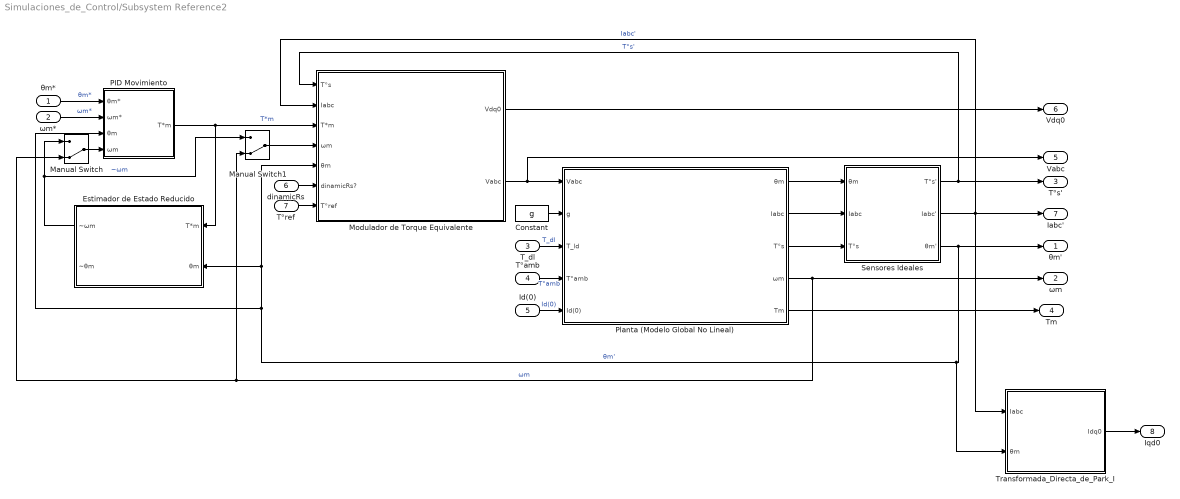
== system Simulaciones_de_Control/Subsystem Reference2 ==
  θm* : Inport
  ωm* : Inport  Port=2
  T_dl : Inport  Port=3
  T°amb : Inport  Port=4
  Id(0) : Inport  Port=5
  dinamicRs : Inport  Port=6
  T°ref : Inport  Port=7
  Constant : Constant  Value=g
  Estimador de Estado Reducido : Subsystem
  Manual Switch : ManualSwitch  CurrentSetting=0
  Manual Switch1 : ManualSwitch  CurrentSetting=0
  Modulador de Torque Equivalente : Subsystem
      settings: PortSchema="{\"entries\":[{\"content\":{\"sides\":[{\"content\":{\"connectorIds\":[\"In1\",\"In3\",\"In5\",\"In2\",\"In4\",\"In6\",\"In7\"]},\"type\":\"ConnectorPlacement.EquallySpacedRectSide\",\"uuid\":\"ea9ad4ab-f607-4d37-9442-85f6cfda2486\"},{\"content\":{\"connectorIds\":[\"Out2\",\"Out1\"],\"side\":\"RIGHT\"},\"type\":\"ConnectorPlacement.EquallySpacedRectSide\",\"uuid\":\"696b5fe5-1f6c-4fc9-932e-86b56d49996f\"},{\"content\":{\"side\":\"TOP\"},\"type\":\"ConnectorPlacement.EquallySpacedRectSide\",\"uuid\":\"45e3ac4c-5a2f-4a79-9454-e497b07295c7\"}]},\"type\":\"ConnectorPlacement.EquallySpacedConnector\",\"uuid\":\"ad401c21-3c60-4ab4-96eb-f449fc93609a\"}],\"packageUris\":[\"http://schema.mathworks.com/mf0/Connector/R2020b\"],\"version\":\"1.0\"}"
  PID Movimiento : Subsystem
      settings: PortSchema="{\"entries\":[{\"content\":{\"sides\":[{\"content\":{\"connectorIds\":[\"In3\",\"In4\",\"In2\",\"In1\"]},\"type\":\"ConnectorPlacement.EquallySpacedRectSide\",\"uuid\":\"99b9ec4b-f651-40ed-8a16-085c2c4ac88d\"},{\"content\":{\"connectorIds\":[\"Out1\"],\"side\":\"RIGHT\"},\"type\":\"ConnectorPlacement.EquallySpacedRectSide\",\"uuid\":\"009a9369-fd86-4ac2-a423-7c7f1491457b\"},{\"content\":{\"side\":\"TOP\"},\"type\":\"ConnectorPlacement.EquallySpacedRectSide\",\"uuid\":\"0bc889a5-9100-482e-a11a-4c36993d76f7\"}]},\"type\":\"ConnectorPlacement.EquallySpacedConnector\",\"uuid\":\"de270b8a-8a15-46e7-87f3-10db7988a399\"}],\"packageUris\":[\"http://schema.mathworks.com/mf0/Connector/R2020b\"],\"version\":\"1.0\"}"
  Planta (Modelo Global No Lineal) : Subsystem
      settings: PortSchema="{\"entries\":[{\"content\":{\"sides\":[{\"content\":{\"connectorIds\":[\"In1\",\"In3\",\"In2\",\"In4\",\"In5\"]},\"type\":\"ConnectorPlacement.EquallySpacedRectSide\",\"uuid\":\"3481abf0-b0cb-49f6-b93f-5a31fbfa4119\"},{\"content\":{\"connectorIds\":[\"Out1\",\"Out2\",\"Out3\",\"Out4\",\"Out5\"],\"side\":\"RIGHT\"},\"type\":\"ConnectorPlacement.EquallySpacedRectSide\",\"uuid\":\"81dbc61e-d5f3-4edc-bc73-ec3d6160a008\"},{\"content\":{\"side\":\"TOP\"},\"type\":\"ConnectorPlacement.EquallySpacedRectSide\",\"uuid\":\"48e37594-92fb-4835-b4aa-9211b8b6a309\"}]},\"type\":\"ConnectorPlacement.EquallySpacedConnector\",\"uuid\":\"6c32b8e1-5803-41f4-af4e-ba3a494349ba\"}],\"packageUris\":[\"http://schema.mathworks.com/mf0/Connector/R2020b\"],\"version\":\"1.0\"}"
  Sensores Ideales : Subsystem
      settings: PortSchema="{\"entries\":[{\"content\":{\"sides\":[{\"content\":{\"connectorIds\":[\"In1\",\"In2\",\"In3\"]},\"type\":\"ConnectorPlacement.EquallySpacedRectSide\",\"uuid\":\"f4bb6189-c8cb-4d3e-a45f-895d59b6a7f9\"},{\"content\":{\"connectorIds\":[\"Out3\",\"Out2\",\"Out1\"],\"side\":\"RIGHT\"},\"type\":\"ConnectorPlacement.EquallySpacedRectSide\",\"uuid\":\"4fe23da4-d7b3-4116-8a5c-3a889a14c1ed\"},{\"content\":{\"side\":\"TOP\"},\"type\":\"ConnectorPlacement.EquallySpacedRectSide\",\"uuid\":\"3a675bb7-2a54-45fb-91cd-5f3dc1d0d742\"}]},\"type\":\"ConnectorPlacement.EquallySpacedConnector\",\"uuid\":\"fa703284-8060-4ab8-a349-fe5cb05f502a\"}],\"packageUris\":[\"http://schema.mathworks.com/mf0/Connector/R2020b\"],\"version\":\"1.0\"}"
  Transformada_Directa_de_Park_I : Subsystem
  θm' : Outport
  ωm : Outport  Port=2
  T°s' : Outport  Port=3
  Tm : Outport  Port=4
  Vabc : Outport  Port=5  OutDataTypeStr=Bus: Vabc
  Vdq0 : Outport  Port=6  OutDataTypeStr=Bus: Vdq0
  Iabc' : Outport  Port=7  OutDataTypeStr=Bus: Iabc
  Iqd0 : Outport  Port=8  OutDataTypeStr=Bus: Idq0
  wires:
  Transformada_Directa_de_Park_I/1(Idq0) -> Iqd0/1
  T°ref/1 -> Modulador de Torque Equivalente/7(T°ref)
  dinamicRs/1 -> Modulador de Torque Equivalente/6(dinamicRs?)
  Modulador de Torque Equivalente/2(Vdq0) -> Vdq0/1
  Planta (Modelo Global No Lineal)/5(Tm) -> Tm/1
  T_dl/1 -> Planta (Modelo Global No Lineal)/2(T_ld)  "T_dl"
  T°amb/1 -> Planta (Modelo Global No Lineal)/4(T°amb)  "T°amb"
  Id(0)/1 -> Planta (Modelo Global No Lineal)/5(Id(0))  "Id(0)"
  Constant/1 -> Planta (Modelo Global No Lineal)/3(g)
  Sensores Ideales/3(T°s') -> Modulador de Torque Equivalente/1(T°s), T°s'/1  "T°s'"
  Sensores Ideales/2(Iabc') -> Iabc'/1, Modulador de Torque Equivalente/3(Iabc), Transformada_Directa_de_Park_I/1(Iabc)  "Iabc'"
  Planta (Modelo Global No Lineal)/3(T°s) -> Sensores Ideales/3(T°s)
  Modulador de Torque Equivalente/1(Vabc) -> Vabc/1, Planta (Modelo Global No Lineal)/1(Vabc)
  Planta (Modelo Global No Lineal)/2(Iabc) -> Sensores Ideales/2(Iabc)
  Sensores Ideales/1(θm') -> PID Movimiento/2(θm), Estimador de Estado Reducido/2(θm), Modulador de Torque Equivalente/4(θm), Transformada_Directa_de_Park_I/2(θm), θm'/1  "θm'"
  Planta (Modelo Global No Lineal)/1(θm) -> Sensores Ideales/1(θm)
  θm*/1 -> PID Movimiento/3(θm*)  "θm*"
  PID Movimiento/1(T*m) -> Estimador de Estado Reducido/1(T*m), Modulador de Torque Equivalente/5(T*m)  "T*m"
  Estimador de Estado Reducido/1(~ωm) -> Manual Switch1/1, Manual Switch/1  "~ωm"
  ωm*/1 -> PID Movimiento/4(ωm*)  "ωm*"
  Planta (Modelo Global No Lineal)/4(ωm) -> Manual Switch/2, Manual Switch1/2, ωm/1  "ωm"
  Manual Switch/1 -> PID Movimiento/1(ωm)
  Manual Switch1/1 -> Modulador de Torque Equivalente/2(ωm)

== system Simulaciones_de_Control/Subsystem Reference3 ==
  q* : Inport
  dq* : Inport  Port=2
  set : Inport  Port=3
  Gain : Gain  Gain=r
  Gain1 : Gain  Gain=r
  Integrator : Integrator  ExternalReset=level  InitialConditionSource=external
  Selector : RelationalOperator  Operator=>  OutDataTypeStr=boolean  RndMeth=Simplest  InputSameDT=off
  Switch : Switch  Criteria=u2 ~= 0  SaturateOnIntegerOverflow=off  InputSameDT=off
  Umbral : Constant  Value=0.5
  θm* : Outport
  ωm* : Outport  Port=2
  wires:
  q*/1 -> Gain/1
  dq*/1 -> Gain1/1
  set/1 -> Selector/1
  Umbral/1 -> Selector/2
  Gain/1 -> Integrator/3, Switch/1
  Selector/1 -> Integrator/2, Switch/2
  Gain1/1 -> Integrator/1, ωm*/1
  Integrator/1 -> Switch/3
  Switch/1 -> θm*/1

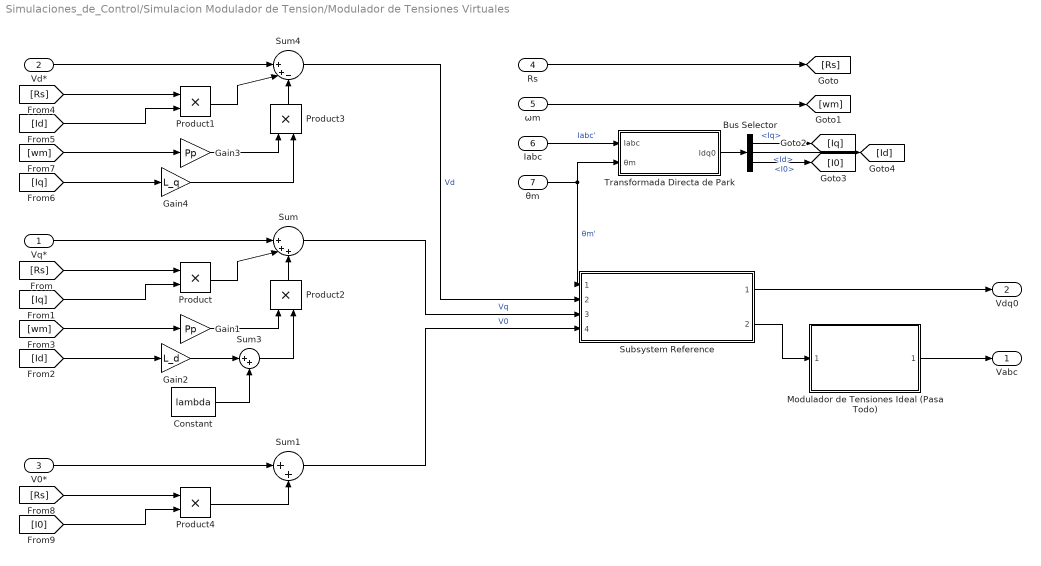
== system Simulaciones_de_Control/Simulacion Modulador de Tension/Modulador de Tensiones Virtuales ==
  Vq* : Inport
  Vd* : Inport  Port=2
  V0* : Inport  Port=3
  Rs : Inport  Port=4
  ωm : Inport  Port=5
  Iabc : Inport  Port=6
  θm : Inport  Port=7
  Bus Selector : BusSelector  OutputSignals=Iq,Id,I0
  Constant : Constant  Value=lambda
  Gain1 : Gain  Gain=Pp
  Gain2 : Gain  Gain=L_d
  Gain3 : Gain  Gain=Pp
  Gain4 : Gain  Gain=L_q
  Modulador de Tensiones Ideal (Pasa Todo) : Subsystem  ReferencedSubsystem=Inversor_Ideal
  Product{,1..4} (5 alike) : Product
  Subsystem Reference : Subsystem  ReferencedSubsystem=Transformada_Inversa_de_Park_V
  Sum : Sum  Inputs=||+++
  Sum1 : Sum  Inputs=|++
  Sum3 : Sum  Inputs=|++
  Sum4 : Sum  Inputs=||++-
  Transformada Directa de Park : Subsystem
  Vabc : Outport
  Vdq0 : Outport  Port=2
  wires:
  Product4/1 -> Sum1/2
  V0*/1 -> Sum1/1
  [Rs] -> Product4/1
  [I0] -> Product4/2
  [Id] -> Product1/2
  Product3/1 -> Sum4/3
  Gain4/1 -> Product3/2
  Vd*/1 -> Sum4/1
  [Rs] -> Product1/1
  Gain3/1 -> Product3/1
  [Iq] -> Gain4/1
  Product1/1 -> Sum4/2
  [wm] -> Gain3/1
  [Iq] -> Product/2
  Gain1/1 -> Product2/1
  Sum3/1 -> Product2/2
  [wm] -> Gain1/1
  Product2/1 -> Sum/3
  Gain2/1 -> Sum3/1
  [Id] -> Gain2/1
  Constant/1 -> Sum3/2
  Product/1 -> Sum/2
  [Rs] -> Product/1
  Vq*/1 -> Sum/1
  Bus Selector/2 -> [Id]  "<Id>"
  Bus Selector/3 -> [I0]  "<I0>"
  Bus Selector/1 -> [Iq]  "<Iq>"
  ωm/1 -> [wm]
  Rs/1 -> [Rs]
  Subsystem Reference/2 -> Modulador de Tensiones Ideal (Pasa Todo)/1
  Modulador de Tensiones Ideal (Pasa Todo)/1 -> Vabc/1
  θm/1 -> Subsystem Reference/1, Transformada Directa de Park/2(θm)  "θm'"
  Transformada Directa de Park/1(Idq0) -> Bus Selector/1
  Iabc/1 -> Transformada Directa de Park/1(Iabc)  "Iabc'"
  Subsystem Reference/1 -> Vdq0/1
  Sum4/1 -> Subsystem Reference/2  "Vd"
  Sum/1 -> Subsystem Reference/3  "Vq"
  Sum1/1 -> Subsystem Reference/4  "V0"

== system Simulaciones_de_Control/Simulacion Modulador de Tension/Planta (Modelo Global No Lineal) ==
  note: Sistema Global No Lineal
  Vabc : Inport  OutDataTypeStr=Bus: Vabc
  T_ld : Inport  Port=2
  g : Inport  Port=3
  T°amb : Inport  Port=4
  Id(0) : Inport  Port=5
  Bus Selector : BusSelector  OutputSignals=Vd,Vq,V0
  Gain : Gain  Gain=Pp
  Subsistema Electromagnetico : Subsystem
  Subsistema Mecanico Equivalente : Subsystem
  Subsistema Termico : Subsystem
  Transformada Directa de Park : Subsystem  ReferencedSubsystem=Transformada_Directa_de_Park_V
  Transformada Inversa de Park : Subsystem  ReferencedSubsystem=Transformada_Inversa_de_Park_I
  θm : Outport
  Iabc : Outport  Port=2  OutDataTypeStr=Bus: Iabc
  T°s : Outport  Port=3
  ωm : Outport  Port=4
  Tm : Outport  Port=5
  wires:
  Id(0)/1 -> Subsistema Electromagnetico/6(Id(0))
  Transformada Inversa de Park/1 -> Iabc/1  "Iabc"
  Bus Selector/3 -> Subsistema Electromagnetico/5(V0)  "<V0>"
  Bus Selector/2 -> Subsistema Electromagnetico/4(Vq)  "<Vq>"
  Bus Selector/1 -> Subsistema Electromagnetico/3(Vd)  "<Vd>"
  Transformada Directa de Park/1 -> Bus Selector/1
  g/1 -> Subsistema Mecanico Equivalente/3(g)
  T°amb/1 -> Subsistema Termico/2(T°amb)
  Vabc/1 -> Transformada Directa de Park/1
  T_ld/1 -> Subsistema Mecanico Equivalente/2(T_ld)
  Gain/1 -> Subsistema Electromagnetico/2(ωr)
  Subsistema Termico/1(R_s) -> Subsistema Electromagnetico/1(R_s)
  Subsistema Electromagnetico/2(T_m) -> Tm/1, Subsistema Mecanico Equivalente/1(T_m)  "Tm"
  Subsistema Mecanico Equivalente/2(θm) -> θm/1, Transformada Inversa de Park/2, Transformada Directa de Park/2  "θm"
  Subsistema Mecanico Equivalente/1(ωm) -> ωm/1, Gain/1  "ωm"
  Subsistema Electromagnetico/1(Idq0) -> Transformada Inversa de Park/1, Subsistema Termico/1(Idq0)  "Idq0"
  Subsistema Termico/2(T°s) -> T°s/1  "T°s"

== system Simulaciones_de_Control/Simulacion Modulador de Tension/Sensores Ideales ==
  note: RTD
  note: Amperimetros
  note: Encoder
  θm : Inport
  Iabc : Inport  Port=2
  T°s : Inport  Port=3
  Bus Creator : BusCreator  Inputs=3
  Bus Selector : BusSelector  OutputSignals=Ia,Ib,Ic
  Gain{,1..4} (5 alike) : Gain
  θm' : Outport
  Iabc' : Outport  Port=2
  T°s' : Outport  Port=3
  wires:
  Gain3/1 -> Bus Creator/3  "Ic"
  Gain1/1 -> Bus Creator/1  "Ia"
  Gain2/1 -> Bus Creator/2  "Ib"
  Bus Selector/3 -> Gain3/1  "<Ic>"
  Bus Selector/2 -> Gain2/1  "<Ib>"
  Bus Selector/1 -> Gain1/1  "<Ia>"
  Iabc/1 -> Bus Selector/1
  Bus Creator/1 -> Iabc'/1
  Gain4/1 -> T°s'/1
  T°s/1 -> Gain4/1
  Gain/1 -> θm'/1
  θm/1 -> Gain/1

== system Simulaciones_de_Control/Simulacion Modulador de Tension/Subsystem ==
  T°s : Inport
  Constant1 : Constant  Value=T_sREF
  Constant2 : Constant
  Gain5 : Gain  Gain=alpha_Cu
  Gain6 : Gain  Gain=R_sREF
  Sum3 : Sum  Inputs=+-|
  Sum4 : Sum  Inputs=|++
  R_s : Outport
  wires:
  Sum3/1 -> Gain5/1
  Sum4/1 -> Gain6/1
  Constant2/1 -> Sum4/2
  Constant1/1 -> Sum3/2
  Gain6/1 -> R_s/1  "R_s"
  Gain5/1 -> Sum4/1
  T°s/1 -> Sum3/1

== system Simulaciones_de_Control/Simulacion Modulador de Tension/Transformada_Directa_de_Park_I ==
  Iabc : Inport  OutDataTypeStr=Bus: Iabc
  θm : Inport  Port=2
  Bus Creator : BusCreator  Inputs=3
  Demux : Demux  Outputs=3
  Gain3 : Gain  Gain=Pp
  Park Transform : eeTransforms/Park Transform  AxisAlignment=Q-axis  PowerInvariant=off
      settings: LibrarySourceBlock=|
      | ee_sl_lib/Mathematical
      | Transforms/Park Transform
  Idq0 : Outport  OutDataTypeStr=Bus: Idq0
  wires:
  Gain3/1 -> Park Transform/2
  Park Transform/1 -> Demux/1  "Idq0"
  Demux/1 -> Bus Creator/1  "Id"
  Demux/3 -> Bus Creator/3  "I0"
  Demux/2 -> Bus Creator/2  "Iq"
  Bus Creator/1 -> Idq0/1
  Iabc/1 -> Park Transform/1
  θm/1 -> Gain3/1

== system Simulaciones_de_Control/Subsystem Reference/Modulador de Torque Equivalente ==
  T°s : Inport
  ωm : Inport  Port=2
  Iabc : Inport  Port=3
  θm : Inport  Port=4
  T*m : Inport  Port=5
  dinamicRs? : Inport  Port=6
  T°ref : Inport  Port=7
  Constant1 : Constant  Value=g
  Constant2 : Constant  Value=T_sREF
  Constant3 : Constant
  Gain : Gain  Gain=alpha_Cu
  Gain1 : Gain  Gain=R_sREF
  Ground : Ground
  Lazo de Control de Corrientes Virtuales : Subsystem  ReferencedSubsystem=Lazo_Corrientes
      settings: PortSchema="{\"entries\":[{\"content\":{\"sides\":[{\"content\":{\"connectorIds\":[\"In2\",\"In3\",\"In1\",\"In4\",\"In5\"]},\"type\":\"ConnectorPlacement.EquallySpacedRectSide\",\"uuid\":\"7378df2b-1b9c-42cd-9ef6-9bfa4de31228\"},{\"content\":{\"connectorIds\":[\"Out2\",\"Out1\",\"Out3\"],\"side\":\"RIGHT\"},\"type\":\"ConnectorPlacement.EquallySpacedRectSide\",\"uuid\":\"75ac4e09-b611-4ee2-aa1e-16791f3f98b8\"},{\"content\":{\"side\":\"TOP\"},\"type\":\"ConnectorPlacement.EquallySpacedRectSide\",\"uuid\":\"c32b7829-5b6a-417b-8aae-eaa4caf59bef\"}]},\"type\":\"ConnectorPlacement.EquallySpacedConnector\",\"uuid\":\"1d84f5ff-db01-492a-bfe1-22065b3eebb0\"}],\"packageUris\":[\"http://schema.mathworks.com/mf0/Connector/R2020b\"],\"version\":\"1.0\"}"
  Modulador de Tensiones Virtuales : Subsystem  ReferencedSubsystem=Modulador_Tensiones
      settings: PortSchema="{\"entries\":[{\"content\":{\"sides\":[{\"content\":{\"connectorIds\":[\"In2\",\"In1\",\"In3\",\"In6\",\"In7\",\"In5\",\"In4\"]},\"type\":\"ConnectorPlacement.EquallySpacedRectSide\",\"uuid\":\"561a625a-719f-47d4-85d3-a88e423068dd\"},{\"content\":{\"connectorIds\":[\"Out2\",\"Out1\"],\"side\":\"RIGHT\"},\"type\":\"ConnectorPlacement.EquallySpacedRectSide\",\"uuid\":\"c1cdd74a-6c1d-470e-a6ac-8d72e83b5cc5\"},{\"content\":{\"side\":\"TOP\"},\"type\":\"ConnectorPlacement.EquallySpacedRectSide\",\"uuid\":\"c5935c6f-534c-46b9-aa64-6d6dabbbb210\"}]},\"type\":\"ConnectorPlacement.EquallySpacedConnector\",\"uuid\":\"b0debde9-6e18-4e06-b0c4-28c9c51e472d\"}],\"packageUris\":[\"http://schema.mathworks.com/mf0/Connector/R2020b\"],\"version\":\"1.0\"}"
  Modulador y Compensación de Torque : Subsystem  ReferencedSubsystem=Lazo_Torque
      settings: PortSchema="{\"entries\":[{\"content\":{\"sides\":[{\"content\":{\"connectorIds\":[\"In5\",\"In1\",\"In2\",\"In3\",\"In4\"]},\"type\":\"ConnectorPlacement.EquallySpacedRectSide\",\"uuid\":\"ea9ad4ab-f607-4d37-9442-85f6cfda2486\"},{\"content\":{\"connectorIds\":[\"Out1\"],\"side\":\"RIGHT\"},\"type\":\"ConnectorPlacement.EquallySpacedRectSide\",\"uuid\":\"696b5fe5-1f6c-4fc9-932e-86b56d49996f\"},{\"content\":{\"side\":\"TOP\"},\"type\":\"ConnectorPlacement.EquallySpacedRectSide\",\"uuid\":\"45e3ac4c-5a2f-4a79-9454-e497b07295c7\"}]},\"type\":\"ConnectorPlacement.EquallySpacedConnector\",\"uuid\":\"ad401c21-3c60-4ab4-96eb-f449fc93609a\"}],\"packageUris\":[\"http://schema.mathworks.com/mf0/Connector/R2020b\"],\"version\":\"1.0\"}"
  Subsystem : Subsystem
  Sum : Sum  Inputs=|+-
  Sum1 : Sum  Inputs=|++
  Switch : Switch  Criteria=u2 > Threshold  SaturateOnIntegerOverflow=off  InputSameDT=off
  Vabc : Outport
  Vdq0 : Outport  Port=2
  wires:
  Lazo de Control de Corrientes Virtuales/1 -> Modulador de Tensiones Virtuales/1
  Lazo de Control de Corrientes Virtuales/2 -> Modulador de Tensiones Virtuales/2
  Lazo de Control de Corrientes Virtuales/3 -> Modulador de Tensiones Virtuales/3
  Modulador y Compensación de Torque/1 -> Lazo de Control de Corrientes Virtuales/1
  T*m/1 -> Modulador y Compensación de Torque/1
  θm/1 -> Modulador de Tensiones Virtuales/7, Lazo de Control de Corrientes Virtuales/5, Modulador y Compensación de Torque/3  "θm"
  ωm/1 -> Modulador de Tensiones Virtuales/5, Modulador y Compensación de Torque/4  "ωm"
  Modulador de Tensiones Virtuales/1 -> Vabc/1
  Ground/1 -> Lazo de Control de Corrientes Virtuales/2, Lazo de Control de Corrientes Virtuales/3
  Iabc/1 -> Modulador de Tensiones Virtuales/6, Lazo de Control de Corrientes Virtuales/4, Modulador y Compensación de Torque/2  "Iabc"
  T°s/1 -> Subsystem/1(T°s)
  Subsystem/1(R_s) -> Switch/1  "Rs"
  dinamicRs?/1 -> Switch/2  "True_False"
  Switch/1 -> Modulador de Tensiones Virtuales/4  "Rs"
  Gain1/1 -> Switch/3
  Modulador de Tensiones Virtuales/2 -> Vdq0/1
  Constant1/1 -> Modulador y Compensación de Torque/5
  T°ref/1 -> Sum/1
  Constant2/1 -> Sum/2
  Sum/1 -> Gain/1
  Gain/1 -> Sum1/1
  Constant3/1 -> Sum1/2
  Sum1/1 -> Gain1/1

== system Simulaciones_de_Control/Subsystem Reference/Planta (Modelo Global No Lineal) ==
  note: Sistema Global No Lineal
  Vabc : Inport  OutDataTypeStr=Bus: Vabc
  T_ld : Inport  Port=2
  g : Inport  Port=3
  T°amb : Inport  Port=4
  Id(0) : Inport  Port=5
  Bus Selector : BusSelector  OutputSignals=Vd,Vq,V0
  Gain : Gain  Gain=Pp
  Subsistema Electromagnetico : Subsystem
  Subsistema Mecanico Equivalente : Subsystem
  Subsistema Termico : Subsystem
  Transformada Directa de Park : Subsystem
  Transformada Inversa de Park : Subsystem  ReferencedSubsystem=Transformada_Inversa_de_Park_I
  θm : Outport
  Iabc : Outport  Port=2  OutDataTypeStr=Bus: Iabc
  T°s : Outport  Port=3
  ωm : Outport  Port=4
  Tm : Outport  Port=5
  wires:
  Subsistema Termico/2(T°s) -> T°s/1  "T°s"
  Subsistema Electromagnetico/1(Idq0) -> Subsistema Termico/1(Idq0), Transformada Inversa de Park/1  "Idq0"
  Subsistema Mecanico Equivalente/1(ωm) -> Gain/1, ωm/1  "ωm"
  Subsistema Mecanico Equivalente/2(θm) -> Transformada Directa de Park/2(θm), Transformada Inversa de Park/2, θm/1  "θm"
  Subsistema Electromagnetico/2(T_m) -> Subsistema Mecanico Equivalente/1(T_m), Tm/1  "Tm"
  Subsistema Termico/1(R_s) -> Subsistema Electromagnetico/1(R_s)
  Gain/1 -> Subsistema Electromagnetico/2(ωr)
  T_ld/1 -> Subsistema Mecanico Equivalente/2(T_ld)
  Vabc/1 -> Transformada Directa de Park/1(Vabc)
  T°amb/1 -> Subsistema Termico/2(T°amb)
  g/1 -> Subsistema Mecanico Equivalente/3(g)
  Transformada Directa de Park/1(Vdq0) -> Bus Selector/1
  Bus Selector/1 -> Subsistema Electromagnetico/3(Vd)  "<Vd>"
  Bus Selector/2 -> Subsistema Electromagnetico/4(Vq)  "<Vq>"
  Bus Selector/3 -> Subsistema Electromagnetico/5(V0)  "<V0>"
  Transformada Inversa de Park/1 -> Iabc/1  "Iabc"
  Id(0)/1 -> Subsistema Electromagnetico/6(Id(0))

== system Simulaciones_de_Control/Subsystem Reference/Sensores Ideales ==
  note: Encoder
  note: Amperimetros
  note: RTD
  θm : Inport
  Iabc : Inport  Port=2
  T°s : Inport  Port=3
  Bus Creator : BusCreator  Inputs=3
  Bus Selector : BusSelector  OutputSignals=Ia,Ib,Ic
  Gain{,1..4} (5 alike) : Gain
  θm' : Outport
  Iabc' : Outport  Port=2
  T°s' : Outport  Port=3
  wires:
  θm/1 -> Gain/1
  Gain/1 -> θm'/1
  T°s/1 -> Gain4/1
  Gain4/1 -> T°s'/1
  Bus Creator/1 -> Iabc'/1
  Iabc/1 -> Bus Selector/1
  Bus Selector/1 -> Gain1/1  "<Ia>"
  Bus Selector/2 -> Gain2/1  "<Ib>"
  Bus Selector/3 -> Gain3/1  "<Ic>"
  Gain2/1 -> Bus Creator/2  "Ib"
  Gain1/1 -> Bus Creator/1  "Ia"
  Gain3/1 -> Bus Creator/3  "Ic"

== system Simulaciones_de_Control/Subsystem Reference/Transformada_Directa_de_Park_I ==
  Iabc : Inport  OutDataTypeStr=Bus: Iabc
  θm : Inport  Port=2
  Ancho_abc : SignalSpecification  Dimensions=3
  Bus Creator : BusCreator  Inputs=3
  Bus to Vector : BusToVector
  Demux : Demux  Outputs=3
  Gain3 : Gain  Gain=Pp
  Park Transform : eeTransforms/Park Transform  AxisAlignment=Q-axis  PowerInvariant=off
      settings: LibrarySourceBlock=|
      | ee_sl_lib/Mathematical
      | Transforms/Park Transform
  Idq0 : Outport  OutDataTypeStr=Bus: Idq0
  wires:
  Gain3/1 -> Park Transform/2
  Park Transform/1 -> Demux/1  "Idq0"
  Demux/1 -> Bus Creator/1  "Id"
  Demux/3 -> Bus Creator/3  "I0"
  Demux/2 -> Bus Creator/2  "Iq"
  Bus Creator/1 -> Idq0/1
  Iabc/1 -> Bus to Vector/1
  θm/1 -> Gain3/1
  Bus to Vector/1 -> Ancho_abc/1
  Ancho_abc/1 -> Park Transform/1

== system Simulaciones_de_Control/Subsystem Reference1/Modulador de Tensiones ==
  Vabc* : Inport
  Bus Creator : BusCreator  Inputs=3
  Demux : Demux  Outputs=3
  Gain1 : Gain
  Gain2 : Gain
  Gain3 : Gain
  Vabc : Outport
  wires:
  Bus Creator/1 -> Vabc/1
  Demux/3 -> Gain3/1
  Demux/1 -> Gain1/1
  Vabc*/1 -> Demux/1
  Demux/2 -> Gain2/1
  Gain1/1 -> Bus Creator/1  "Va"
  Gain3/1 -> Bus Creator/3  "Vc"
  Gain2/1 -> Bus Creator/2  "Vb"

== system Simulaciones_de_Control/Subsystem Reference1/Sensores ==
  note: Encoder
  note: Amperimetros
  note: RTD
  θm : Inport
  Iabc : Inport  Port=2
  T°s : Inport  Port=3
  Bus Creator : BusCreator  Inputs=3
  Bus Selector : BusSelector  OutputSignals=Ia,Ib,Ic
  Gain{,1..4} (5 alike) : Gain
  θm' : Outport
  Iabc' : Outport  Port=2
  T°s' : Outport  Port=3
  wires:
  θm/1 -> Gain/1
  Gain/1 -> θm'/1
  T°s/1 -> Gain4/1
  Gain4/1 -> T°s'/1
  Bus Creator/1 -> Iabc'/1
  Iabc/1 -> Bus Selector/1
  Bus Selector/1 -> Gain1/1  "<Ia>"
  Bus Selector/2 -> Gain2/1  "<Ib>"
  Bus Selector/3 -> Gain3/1  "<Ic>"
  Gain2/1 -> Bus Creator/2  "Ib"
  Gain1/1 -> Bus Creator/1  "Ia"
  Gain3/1 -> Bus Creator/3  "Ic"

== system Simulaciones_de_Control/Subsystem Reference1/Sistema Global No Lineal ==
  note: Sistema Global No Lineal
  Vabc : Inport  OutDataTypeStr=Bus: Vabc
  T_ld : Inport  Port=2
  g : Inport  Port=3
  T°amb : Inport  Port=4
  Id(0) : Inport  Port=5
  Bus Selector : BusSelector  OutputSignals=Vd,Vq,V0
  Gain : Gain  Gain=Pp
  Subsistema Electromagnetico : Subsystem
  Subsistema Mecanico Equivalente : Subsystem
  Subsistema Termico : Subsystem
  Transformada Directa de Park : Subsystem
  Transformada Inversa de Park : Subsystem
  θm : Outport
  Iabc : Outport  Port=2  OutDataTypeStr=Bus: Iabc
  T°s : Outport  Port=3
  ωm : Outport  Port=4
  Tm : Outport  Port=5
  wires:
  Subsistema Termico/2(T°s) -> T°s/1  "T°s"
  Subsistema Electromagnetico/1(Idq0) -> Subsistema Termico/1(Idq0), Transformada Inversa de Park/1(Idq0)  "Idq0"
  Subsistema Mecanico Equivalente/1(ωm) -> Gain/1, ωm/1  "ωm"
  Subsistema Mecanico Equivalente/2(θm) -> Transformada Directa de Park/2(θm), Transformada Inversa de Park/2(θm), θm/1  "θm"
  Subsistema Electromagnetico/2(T_m) -> Subsistema Mecanico Equivalente/1(T_m), Tm/1  "Tm"
  Subsistema Termico/1(R_s) -> Subsistema Electromagnetico/1(R_s)
  Gain/1 -> Subsistema Electromagnetico/2(ωr)
  T_ld/1 -> Subsistema Mecanico Equivalente/2(T_ld)
  Vabc/1 -> Transformada Directa de Park/1(Vabc)
  T°amb/1 -> Subsistema Termico/2(T°amb)
  g/1 -> Subsistema Mecanico Equivalente/3(g)
  Transformada Directa de Park/1(Vdq0) -> Bus Selector/1
  Bus Selector/1 -> Subsistema Electromagnetico/3(Vd)  "<Vd>"
  Bus Selector/2 -> Subsistema Electromagnetico/4(Vq)  "<Vq>"
  Bus Selector/3 -> Subsistema Electromagnetico/5(V0)  "<V0>"
  Transformada Inversa de Park/1(Iabc) -> Iabc/1  "Iabc"
  Id(0)/1 -> Subsistema Electromagnetico/6(Id(0))

== system Simulaciones_de_Control/Subsystem Reference1/Transformada Directa de Park ==
  Iabc : Inport  OutDataTypeStr=Bus: Iabc
  θm : Inport  Port=2
  Bus Creator : BusCreator  Inputs=3
  Demux : Demux  Outputs=3
  Gain3 : Gain  Gain=Pp
  Park Transform : eeTransforms/Park Transform  AxisAlignment=Q-axis  PowerInvariant=off
      settings: LibrarySourceBlock=|
      | ee_sl_lib/Mathematical
      | Transforms/Park Transform
  Idq0 : Outport  OutDataTypeStr=Bus: Idq0
  wires:
  Gain3/1 -> Park Transform/2
  Park Transform/1 -> Demux/1  "Idq0"
  Demux/1 -> Bus Creator/1  "Id"
  Demux/3 -> Bus Creator/3  "I0"
  Demux/2 -> Bus Creator/2  "Iq"
  Bus Creator/1 -> Idq0/1
  Iabc/1 -> Park Transform/1
  θm/1 -> Gain3/1

== system Simulaciones_de_Control/Subsystem Reference1/Transformada Directa de Park1 ==
  Iabc : Inport  OutDataTypeStr=Bus: Iabc
  θm : Inport  Port=2
  Bus Creator : BusCreator  Inputs=3
  Demux : Demux  Outputs=3
  Gain3 : Gain  Gain=Pp
  Park Transform : eeTransforms/Park Transform  AxisAlignment=Q-axis  PowerInvariant=off
      settings: LibrarySourceBlock=|
      | ee_sl_lib/Mathematical
      | Transforms/Park Transform
  Idq0 : Outport  OutDataTypeStr=Bus: Idq0
  wires:
  Gain3/1 -> Park Transform/2
  Park Transform/1 -> Demux/1  "Idq0"
  Demux/1 -> Bus Creator/1  "Id"
  Demux/3 -> Bus Creator/3  "I0"
  Demux/2 -> Bus Creator/2  "Iq"
  Bus Creator/1 -> Idq0/1
  Iabc/1 -> Park Transform/1
  θm/1 -> Gain3/1
